simulink model "ACFT11_a_121"  (R2026a)
settings: Solver=ode15s  StopTime=2400  FixedStep=0.01  MaxStep=0.05  MinStep=1e-4  AbsTol=1e-4
model workspace (MAT data in the model file):
  op11 = opcond.OperatingPoint
  op11.Model_ = 'ACFT'
  op11.States_(1) = opcond.StatePoint
  op11.States_(1).Nx_ = 1
  op11.States_(1).Block_ = 'ACFT/EqM/BodyRates/p_radps'
  op11.States_(1).StateName_ = 'p_radps'
  op11.States_(1).x_ = -1.51786990083e-19
  op11.States_(2) = opcond.StatePoint
  op11.States_(2).Nx_ = 1
  op11.States_(2).Block_ = 'ACFT/EqM/BodyRates/q_radps'
  op11.States_(2).StateName_ = 'q_radps'
  op11.States_(2).x_ = 1.34070454591e-20
  op11.States_(3) = opcond.StatePoint
  op11.States_(3).Nx_ = 1
  op11.States_(3).Block_ = 'ACFT/EqM/BodyRates/r_radps'
  op11.States_(3).StateName_ = 'r_radps'
  op11.States_(3).x_ = 3.04056373945e-20
  op11.States_(4) = opcond.StatePoint
  op11.States_(4).Nx_ = 1
  op11.States_(4).Block_ = 'ACFT/EqM/BodyVelocities/u_mps'
  op11.States_(4).StateName_ = 'u_mps'
  op11.States_(4).x_ = 221.237928753
  op11.States_(5) = opcond.StatePoint
  op11.States_(5).Nx_ = 1
  op11.States_(5).Block_ = 'ACFT/EqM/BodyVelocities/v_mps'
  op11.States_(5).StateName_ = 'v_mps'
  op11.States_(5).x_ = -6.28259554611e-18
  op11.States_(6) = opcond.StatePoint
  op11.States_(6).Nx_ = 1
  op11.States_(6).Block_ = 'ACFT/EqM/BodyVelocities/w_mps'
  op11.States_(6).StateName_ = 'w_mps'
  op11.States_(6).x_ = 38.749469963
  op11.States_(7) = opcond.StatePoint
  op11.States_(7).Nx_ = 1
  op11.States_(7).Block_ = 'ACFT/EqM/EulerAngles/PHI_rad'
  op11.States_(7).StateName_ = 'PHI_rad'
  op11.States_(7).x_ = 1.38680229931e-18
  op11.States_(8) = opcond.StatePoint
  op11.States_(8).Nx_ = 1
  op11.States_(8).Block_ = 'ACFT/EqM/EulerAngles/PSI_rad'
  op11.States_(8).StateName_ = 'PSI_rad'
  op11.States_(8).x_ = -6.63244493967e-13
  op11.States_(9) = opcond.StatePoint
  op11.States_(9).Nx_ = 1
  op11.States_(9).Block_ = 'ACFT/EqM/EulerAngles/THETA_rad'
  op11.States_(9).StateName_ = 'THETA_rad'
  op11.States_(9).x_ = 0.17338965629
  op11.States_(10) = opcond.StatePoint
  op11.States_(10).Nx_ = 1
  op11.States_(10).Block_ = 'ACFT/EqM/InertialData/XI_m'
  op11.States_(10).StateName_ = 'XI_m'
  op11.States_(10).x_ = -1.46881201642e-12
  op11.States_(11) = opcond.StatePoint
  op11.States_(11).Nx_ = 1
  op11.States_(11).Block_ = 'ACFT/EqM/InertialData/YI_m1'
  op11.States_(11).StateName_ = 'YI_m'
  op11.States_(11).x_ = -2.21671166849e-12
  op11.States_(12) = opcond.StatePoint
  op11.States_(12).Nx_ = 1
  op11.States_(12).Block_ = 'ACFT/EqM/InertialData/ZI_m'
  op11.States_(12).StateName_ = 'ZI_m'
  op11.States_(12).x_ = -9997.44
  op11.Inputs_(1) = opcond.InputPoint
  op11.Inputs_(1).Block_ = 'ACFT/Elevator_deg'
  op11.Inputs_(1).PortWidth_ = 1
  op11.Inputs_(1).PortDimensions_ = [1 1]
  op11.Inputs_(1).u_ = -3.63207180524
  op11.Inputs_(2) = opcond.InputPoint
  op11.Inputs_(2).Block_ = 'ACFT/Aileron_deg'
  op11.Inputs_(2).PortWidth_ = 1
  op11.Inputs_(2).PortDimensions_ = [1 1]
  op11.Inputs_(2).u_ = 2.99398013712e-18
  op11.Inputs_(3) = opcond.InputPoint
  op11.Inputs_(3).Block_ = 'ACFT/Rudder_deg'
  op11.Inputs_(3).PortWidth_ = 1
  op11.Inputs_(3).PortDimensions_ = [1 1]
  op11.Inputs_(4) = opcond.InputPoint
  op11.Inputs_(4).Block_ = 'ACFT/Throttle'
  op11.Inputs_(4).PortWidth_ = 1
  op11.Inputs_(4).PortDimensions_ = [1 1]
  op11.Inputs_(4).u_ = 0.523236061228
  op_trim1 : opcond.OperatingReport (value not decoded)
  op_trim12 : opcond.OperatingReport (value not decoded)
  op_trim15 : opcond.OperatingReport (value not decoded)
  op_trim16 : opcond.OperatingReport (value not decoded)
  op_trim17 : opcond.OperatingReport (value not decoded)
  op_trim18 : opcond.OperatingReport (value not decoded)
  op_trim2 : opcond.OperatingReport (value not decoded)
  op_trim20 : opcond.OperatingReport (value not decoded)
  op_trim21 : opcond.OperatingReport (value not decoded)
  op_trim22 : opcond.OperatingReport (value not decoded)
  op_trim23 : opcond.OperatingReport (value not decoded)
  op_trim24 : opcond.OperatingReport (value not decoded)
  op_trim25 : opcond.OperatingReport (value not decoded)
  op_trim29 : opcond.OperatingReport (value not decoded)
  op_trim3 : opcond.OperatingReport (value not decoded)
  op_trim30 : opcond.OperatingReport (value not decoded)
  op_trim4 : opcond.OperatingReport (value not decoded)
  op_trim40 : opcond.OperatingReport (value not decoded)
  op_trim42 : opcond.OperatingReport (value not decoded)
  op_trim5 : opcond.OperatingReport (value not decoded)
  op_trim50 : opcond.OperatingReport (value not decoded)
  op_trim7 : opcond.OperatingReport (value not decoded)
  op_trim9 : opcond.OperatingReport (value not decoded)
values from neighbouring files (symbols this model uses):
  b = 9.05    [inertiatensor62.m]    (also in setup_bfl_analysis.m; setup_fcs_sim.m; setup_gschedule.m = geom.FCS_b; setup_takeoff_fcs.m)
  c = bar_colors{min(k,numel(bar_colors))}    [analyze_bfl.m]    (also in inertiatensor62.m = 15.55; optimize_indi_gains.m = 15.55; restore_normal_fcs.m = 15.55; run_bfl_sweep.m = 15.55)
  CL_AlphaDot = 0    [inertiatensor62.m]    (also in setup_bfl_analysis.m; setup_fcs_sim.m; setup_takeoff_fcs.m)
  Cm_AlphaDot = 0    [inertiatensor62.m]    (also in setup_bfl_analysis.m; setup_fcs_sim.m; setup_takeoff_fcs.m)
  FCS_aerospike_thrust = 250000.0    (= 250000)    [fcs_params.m]
  FCS_alpha_max = 16.0    (= 16)    [fcs_params.m]
  FCS_bank_max = 45.0    (= 45)    [fcs_params.m]
  FCS_da_max = 20.0    (= 20)    [fcs_params.m]
  FCS_de_max = 25.0    (= 25)    [fcs_params.m]
  FCS_dr_max = 25.0    (= 25)    [fcs_params.m]
  FCS_dt = 0.01    [fcs_params.m]
  FCS_g = 9.80665    [fcs_params.m]
  FCS_Gmin_p = 0.02    [fcs_params.m]
  FCS_Gmin_q = 0.02    [fcs_params.m]
  FCS_Gmin_r = 0.01    [fcs_params.m]
  FCS_h_gnd = 2.24    [fcs_params.m]
  FCS_hdot_max = 30.0    (= 30)    [fcs_params.m]
  FCS_hdot_td = 0.3    [fcs_params.m]
  FCS_Kalpha = 3.0    (= 3)    [fcs_params.m]
  FCS_Kalpha_lim = 2.0    (= 2)    [fcs_params.m]
  FCS_Kbeta = 2.0    (= 2)    [fcs_params.m]
  FCS_Kflare = 1.0    (= 1)    [fcs_params.m]
  FCS_Kgamma = 1.5    [fcs_params.m]
  FCS_Kh = 0.10    (= 0.1)    [fcs_params.m]
  FCS_Knz = 20.0    (= 20)    [fcs_params.m]
  FCS_Kp = 6.0    (= 6)    [fcs_params.m]
  FCS_Kphi = 3.0    (= 3)    [fcs_params.m]
  FCS_Kq = 5.0    (= 5)    [fcs_params.m]
  FCS_Kr = 4.0    (= 4)    [fcs_params.m]
  FCS_Ktheta = 2.0    (= 2)    [fcs_params.m]
  FCS_link_timeout = 1.0    (= 1)    [fcs_params.m]
  FCS_MODE_AUTO = 0    [fcs_params.m]
  FCS_Nfilt = 20.0    (= 20)    [fcs_params.m]
  FCS_Nz_max = 3.0    (= 3)    [fcs_params.m]
  FCS_Nz_min = -1.0    (= -1)    [fcs_params.m]
  FCS_p_max = 60.0    (= 60)    [fcs_params.m]
  FCS_q_max = 15.0    (= 15)    [fcs_params.m]
  FCS_qbar_hi = 6000.0    (= 6000)    [fcs_params.m]
  FCS_qbar_lo = 1000.0    (= 1000)    [fcs_params.m]
  FCS_r_max = 15.0    (= 15)    [fcs_params.m]
  FCS_relight_M_hi = 2.0    (= 2)    [fcs_params.m]
  FCS_relight_M_lo = 0.35    [fcs_params.m]
  FCS_relight_qbar = 3000.0    (= 3000)    [fcs_params.m]
  FCS_stick_detent = 0.03    [fcs_params.m]
  FCS_stick_p_scale = 60.0    (= 60)    [fcs_params.m]
  FCS_stick_q_scale = 15.0    (= 15)    [fcs_params.m]
  FCS_tau_flare = 8.0    (= 8)    [fcs_params.m]
  FCS_TECS_Kep = 0.25    [fcs_params.m]
  FCS_TECS_Ktp = 0.30    (= 0.3)    [fcs_params.m]
  FCS_theta_climb = 12.0    (= 12)    [fcs_params.m]
  FCS_theta_max = 30.0    (= 30)    [fcs_params.m]
  FCS_theta_min = -20.0    (= -20)    [fcs_params.m]
  FCS_theta_trim = 0.0    (= 0)    [fcs_params.m]
  FCS_thr_max = 1.0    (= 1)    [fcs_params.m]
  FCS_thr_min = 0.0    (= 0)    [fcs_params.m]
  FCS_thr_trim = 0.50    (= 0.5)    [fcs_params.m]
  FCS_V_rotate = 94.0    (= 94)    [fcs_params.m]
  FCS_Vmin = 60.0    (= 60)    [fcs_params.m]
  FF_rates = [0.0,              2.5,              5.0,             73.0,             78.0,              0.5]    [fcs_params.m]
  g = 9.80665    [inertiatensor62.m]    (also in setup_bfl_analysis.m; setup_fcs_sim.m; setup_takeoff_fcs.m)
  GS_Gp_tab = Cl_da * (S*b/Ixx)    [setup_gschedule.m]
  GS_Gq_tab = Cm_de * (S*c/Iyy)    [setup_gschedule.m]
  GS_Gr_tab = Cn_dr * (S*b/Izz)    [setup_gschedule.m]
  MASS_fuel_total = MASS_full - MASS_empty - MASS_orbiter    (= 14700)    [fcs_params.m]
  S = 85.25    [inertiatensor62.m]    (also in optimize_indi_gains.m; restore_normal_fcs.m; run_bfl_sweep.m; setup_bfl_analysis.m)
  s = [s, sprintf(' ... (first row only)    [setup_propulsion.m]
  y_cg = 0    [inertiatensor62.m]    (also in setup_bfl_analysis.m; setup_fcs_sim.m; setup_takeoff_fcs.m)
  z_cg = 0.0    (= 0)    [inertiatensor62.m]    (also in setup_bfl_analysis.m; setup_fcs_sim.m; setup_takeoff_fcs.m)
undefined symbols (not defined in the file or in its folder): deg, DiscIntNeverNeededParam, EqM, GS_alpha_cl, GS_alpha_cm, GS_alpha_cn, GS_mach_cl, GS_mach_cm, GS_mach_cn, rad
libraries: aerolibconvert2 x21, simulink x7, aerolibfltsims x3, aerolibanim x1, aerolibatmos2 x1, shareddyn x1
(part 1 of 4)
settings Model: PacingRate=20  Creator=bruno  LastModifiedBy=tejve
settings SolverCC: MaxConsecutiveMinStep=3  ZeroCrossAlgorithm=Adaptive  EnableFixedStepZeroCrossing=on
settings DataIOCC: ExternalInput=takeoff_u  InitialState=getstatestruct(op_trim1)
settings DebuggingCC: MinStepSizeMsg=error  MaskedZcDiagnostic=none  IgnoredZcDiagnostic=none  UnderSpecifiedDimensionMsg=warning

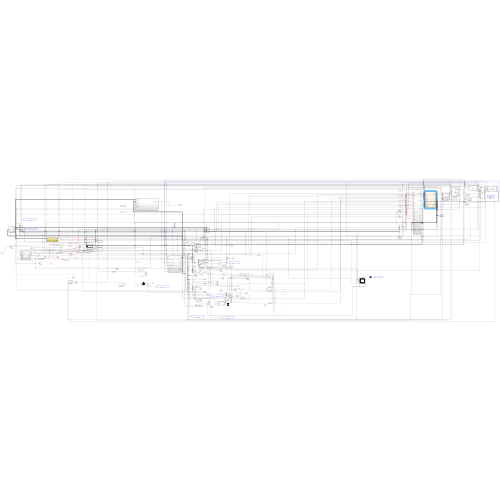
[thumbnail: Simulink's stored preview of the top-level diagram]
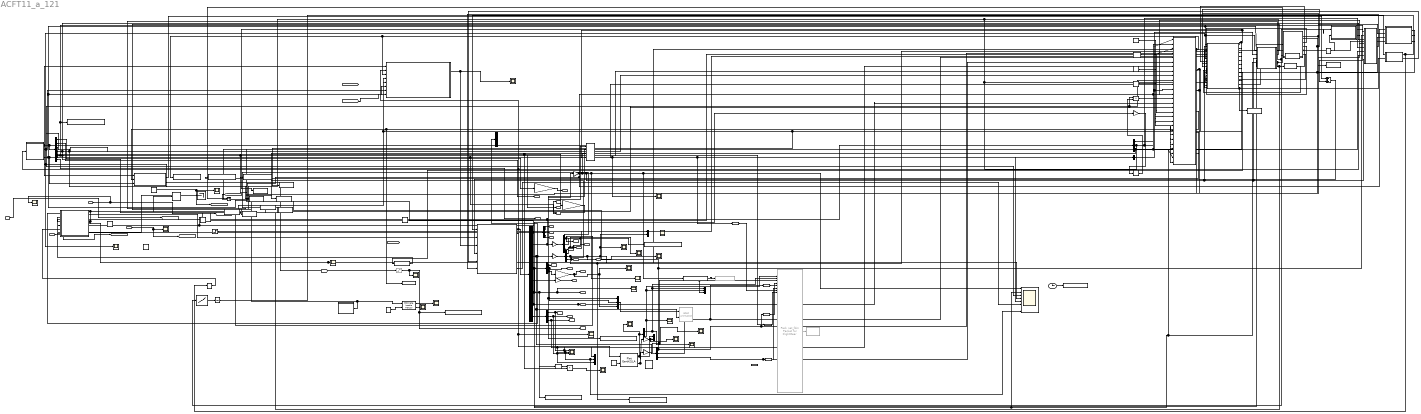
== system ACFT11_a_121 ==
  Elevator_deg : Inport  OutDataTypeStr=double
  Aileron_deg : Inport  Port=2  OutDataTypeStr=double
  Rudder_deg : Inport  Port=3  OutDataTypeStr=double
  Throttle : Inport  Port=4  OutDataTypeStr=double
  6DoF Animation : aerolibanim/6DoF Animation  Commented=on  u1=[0 40000 -20000 20000 -50000 -30000]  u2=0.1  u3=400  u4=[0 0 0]  u5=Fly alongside  u6=[10000 10000 10000]  u7=9  u8=on
  Aerospike : MATLAB Function  TreatAsAtomicUnit=on
  Aerospike_Tmax : Constant  Value=FCS_aerospike_thrust
  Aerovegamidfid : Subsystem  AncestorBlock=Aerodynamic/Aero
  Alt_1000m_trigger : simulink/Logic and Bit Operations/Compare To Constant  relop=>=  const=9999  OutDataTypeStr=boolean
  Angle Conversion : aerolibconvert2/Angle Conversion  IU=deg  OU=rad
  Atmospheric : Subsystem  AncestorBlock=Atmospheric/Atmospheric
  Bus Selector : BusSelector  OutputSignals=CAS_mps,Mach,TAS_mps,Beta_deg,Alpha_deg,AlphaDot_radps
  Bus Selector1 : BusSelector  OutputSignals=VB_mps,BodyRates_radps,EulerAngles_rad,IntertialPosition_m,GroundSpeed_mps,Gamma_deg,Track_deg,LoadFactors
  Cg AS PERCENTGE OF TOTAL LENGTH CREF : Constant  Value=0.6168
  Clock_FCS : Clock
  Constant : Constant  Value=[0,0,0,0,0,0]
  Constant1 : Constant
  Constant2 : Constant  Value=1.2
  Constant3 : Constant  Value=0
  Constant4 : Constant  Value=0
  Data Type Conversion{,1..4,8} (6 alike) : DataTypeConversion  OutDataTypeStr=single  SaturateOnIntegerOverflow=off  RndMeth=Floor
  Demux{,1..5,10} (7 alike) : Demux  Outputs=3
  Demux6 : Demux  Outputs=2
  DtcDesc : DataTypeConversion  OutDataTypeStr=double  SaturateOnIntegerOverflow=off  RndMeth=Floor
  DtcRl : DataTypeConversion  OutDataTypeStr=double  SaturateOnIntegerOverflow=off  RndMeth=Floor
  EqM : Subsystem  AncestorBlock=EqM/EqM
  Estimate Inertia Tensor : shareddyn/Estimate Inertia Tensor  fmass=28500  emass=10800  fI=Inertia  eI=InertiaEmpty  aMode=aMode
      settings: LibrarySourceBlock=|
      | aerolibbdyn/Estimate
      | Inertia Tensor
  Estimation : Subsystem
  FCS : Subsystem
  FCS_RC_age : Constant  Value=0
  FCS_RC_mode : Constant  Value=FCS_MODE_AUTO
  FCS_RC_pitch : Constant  Value=0
  FCS_RC_roll : Constant  Value=0
  FCS_Vz_calc : Product  Inputs=**
  FCS_gamma_d2r : Gain  Gain=pi/180
  FCS_rate_demux : Demux  Outputs=3
  FCS_rho_sel : BusSelector  OutputSignals=rho_kgpm3
  FCS_sin_gamma : Trigonometry
  FfLut : Lookup_n-D  NumberOfTableDimensions=1  BreakpointsForDimension1=[0 1 2 3 4 5]  Table=FF_rates  InterpMethod=Flat  ExtrapMethod=Clip  InternalRulePriority=Speed  RndMeth=Simplest
  Flat Earth to LLA : FlatEarth2LLA  R=6378137  LL0=[36.973889000000000 -25.171111000000000]
  FuelInt : Integrator  UpperSaturationLimit=MASS_fuel_total  LowerSaturationLimit=0
  Gain : Gain
  Gain1 : Gain  Gain=-1
  Gain2 : Gain  Gain=-1
  Generate Run Script1 : aerolibfltsims/Generate Run Script  Architecture=Win64  dataFlow=Send  GeometryModelName=c172p  AirportId=1  RunwayId=1  InitialAltitude=0  InitialHeading=0  OffsetDistance=0  OffsetAzimuth=0  InstallScenery=off  DisableShaders=off  OriginAddress=127.0.0.1  DestinationPort=5502  OriginPort=5505  LocalAddress=127.0.0.1  OutputFileName=tj112.bat  FlightGearBaseDirectory=C:\Program Files\FlightGear 2020.3.2
  GlideCompute : MATLAB Function  TreatAsAtomicUnit=on
  Landing Gear : Subsystem
  ManeuverScope : Scope  NumInputPorts=8
      settings: ActiveDisplayString=8  ActiveDisplayYMinimum=-2.289254531971836  ActiveDisplayYMaximum=5.0402128679995908  DataLoggingVariableName=ScopeData55
  MassModel : MATLAB Function  TreatAsAtomicUnit=on
  MemMass : Memory  InitialCondition=28500
  MissionManager : Stateflow chart  TreatAsAtomicUnit=on
  Mux : Mux  Inputs=2
  Mux1 : Mux  Inputs=3
  Mux3 : Mux  Inputs=3
  Mux4 : Mux  Inputs=2
  Mux7 : Mux  Inputs=3
  Nf_LiftoffScope : Scope
  Pack net_fdm Packet for FlightGear : aerolibfltsims/Pack net_fdm Packet for FlightGear  Commented=on  FlightGearVersion=v2019.1  ShowPositionAttitudeInputs=on  ShowVelocityAccelerationInputs=on  ShowControlSurfacePositionInputs=on  ShowEngineFuelInputs=on  ShowLandingGearInputs=off  ShowEnvironmentInputs=off  SampleTime=-1  packetVersion=24
  Product : Product
  Propulsion : Subsystem  AncestorBlock=Propulsion/Propulsion
  RCS_ctrl : MATLAB Function  TreatAsAtomicUnit=on
  RTB_Guidance : MATLAB Function  TreatAsAtomicUnit=on
  Saturation2 : Saturate  Commented=through  UpperLimit=250000  LowerLimit=0
  Scope{,1..7,10..14,18,20} (15 alike) : Scope
      Scope settings: ActiveDisplayYMinimum=-13.152364949660917  ActiveDisplayYMaximum=60.1028018218888  YLabel=Flight path angle(deg)  DataLoggingVariableName=ScopeData5
      Scope1 settings: ActiveDisplayYMinimum=-1  ActiveDisplayYMaximum=1
      Scope10 settings: ActiveDisplayYMinimum=0.61360792662227759  ActiveDisplayYMaximum=0.63379776950955791  DataLoggingVariableName=ScopeData11
      Scope11 settings: ActiveDisplayYMinimum=-1340.90587  ActiveDisplayYMaximum=11603.05287  DataLoggingVariableName=ScopeData12
      Scope12 settings: ActiveDisplayYMinimum=-623.957  ActiveDisplayYMaximum=5615.613  DataLoggingVariableName=ScopeData13
      Scope13 settings: ActiveDisplayYMinimum=-1  ActiveDisplayYMaximum=1
      Scope14 settings: ActiveDisplayYMinimum=-1.0801678452245245  ActiveDisplayYMaximum=10.282171182560381  DataLoggingVariableName=ScopeData21
      Scope18 settings: ActiveDisplayYMinimum=-1  ActiveDisplayYMaximum=1  DataLoggingVariableName=ScopeData29
      Scope2 settings: ActiveDisplayYMinimum=-1  ActiveDisplayYMaximum=1  DataLoggingVariableName=ScopeData2
      Scope20 settings: ActiveDisplayYMinimum=0.90512395677267277  ActiveDisplayYMaximum=2.9051239567726728  DataLoggingVariableName=ScopeData31
      Scope3 settings: ActiveDisplayYMinimum=-1  ActiveDisplayYMaximum=1  DataLoggingVariableName=ScopeData3
      Scope4 settings: ActiveDisplayYMinimum=-10822.330699949573  ActiveDisplayYMaximum=8964.1397199268285
      Scope5 settings: ActiveDisplayYMinimum=2.6766585887324741  ActiveDisplayYMaximum=69.223535186339291
      Scope6 settings: ActiveDisplayYMinimum=-1.0137729913835152  ActiveDisplayYMaximum=70.044552754707041  DataLoggingVariableName=ScopeData22
      Scope7 settings: ActiveDisplayYMinimum=-35300.079820700717  ActiveDisplayYMaximum=108949.5506916134  DataLoggingVariableName=ScopeData23
  Send net_fdm Packet to FlightGear : aerolibfltsims/Send net_fdm Packet to FlightGear  Commented=on  DestinationIpAddress=127.0.0.1  DestinationPort=5502  LocalIpPort=-1  varLen=off  SampleTime=-1
  Stop_at_1000m : Stop  Commented=on
  TW_Alpha_deg : ToWorkspace  VariableName=TW_Alpha_deg  SampleTime=0.1
  TW_E_spec : ToWorkspace  VariableName=TW_E_spec  SaveFormat=Timeseries  SampleTime=-1
  TW_Gamma_deg : ToWorkspace  VariableName=TW_Gamma_deg  SampleTime=0.1
  TW_Mach : ToWorkspace  VariableName=Machlog  SaveFormat=Timeseries  SampleTime=-1
  TW_MissionPhase : ToWorkspace  VariableName=TW_MissionPhase  SaveFormat=Timeseries  SampleTime=-1
  TW_Ntotal : ToWorkspace  VariableName=TW_Ntotal  SampleTime=0.02
  TW_Phase : ToWorkspace  VariableName=TW_Phase  SampleTime=-1
  TW_TAS_mps : ToWorkspace  VariableName=TW_TAS_mps  SampleTime=0.1
  TW_T_aero : ToWorkspace  VariableName=T_aero  SaveFormat=Timeseries  SampleTime=-1
  TW_Theta_deg : ToWorkspace  VariableName=TW_Theta_deg  SampleTime=0.1
  TW_Throttle : ToWorkspace  VariableName=TW_Throttle  SampleTime=0.02
  TW_Thrust_N : ToWorkspace  VariableName=TW_Thrust_N  SampleTime=0.1
  TW_V : ToWorkspace  VariableName=Vlog  SaveFormat=Timeseries  SampleTime=-1
  TW_Vz_est : ToWorkspace  VariableName=TW_Vz_est  SaveFormat=Timeseries  SampleTime=-1
  TW_X_m : ToWorkspace  VariableName=TW_X_m  SampleTime=0.1
  TW_ail : ToWorkspace  VariableName=TW_ail  SaveFormat=Timeseries  SampleTime=-1
  TW_al : ToWorkspace  VariableName=al_log  SaveFormat=Timeseries  SampleTime=-1
  TW_beta : ToWorkspace  VariableName=TW_beta  SaveFormat=Timeseries  SampleTime=-1
  TW_beta2 : ToWorkspace  VariableName=beta_log  SaveFormat=Timeseries  SampleTime=-1
  TW_brg : ToWorkspace  VariableName=brg_log  SaveFormat=Timeseries  SampleTime=-1
  TW_da : ToWorkspace  VariableName=da_log  SaveFormat=Timeseries  SampleTime=-1
  TW_de : ToWorkspace  VariableName=de_log  SaveFormat=Timeseries  SampleTime=-1
  TW_dr2 : ToWorkspace  VariableName=dr_log  SaveFormat=Timeseries  SampleTime=-1
  TW_elev_cmd : ToWorkspace  VariableName=TW_elev_cmd  SampleTime=-1
  TW_h : ToWorkspace  VariableName=hlog  SaveFormat=Timeseries  SampleTime=-1
  TW_p : ToWorkspace  VariableName=TW_p  SaveFormat=Timeseries  SampleTime=-1
  TW_phase : ToWorkspace  VariableName=phase  SaveFormat=Timeseries  SampleTime=-1
  TW_phi : ToWorkspace  VariableName=phi_log  SaveFormat=Timeseries  SampleTime=-1
  TW_posNED : ToWorkspace  VariableName=TW_posNED  SampleTime=0.02
  TW_prop_mode : ToWorkspace  VariableName=prop_mode  SaveFormat=Timeseries  SampleTime=-1
  TW_psi : ToWorkspace  VariableName=TW_psi  SaveFormat=Timeseries  SampleTime=-1
  TW_q : ToWorkspace  VariableName=q_log2  SaveFormat=Timeseries  SampleTime=-1
  TW_q_deg : ToWorkspace  VariableName=TW_q_deg  SampleTime=0.1
  TW_qbar : ToWorkspace  VariableName=TW_qbar  SaveFormat=Timeseries  SampleTime=-1
  TW_qcmd : ToWorkspace  VariableName=TW_qcmd  SampleTime=-1
  TW_r : ToWorkspace  VariableName=TW_r  SaveFormat=Timeseries  SampleTime=-1
  TW_r2 : ToWorkspace  VariableName=r_log  SaveFormat=Timeseries  SampleTime=-1
  TW_relight_ok : ToWorkspace  VariableName=TW_relight_ok  SaveFormat=Timeseries  SampleTime=-1
  TW_rng : ToWorkspace  VariableName=rng_log  SaveFormat=Timeseries  SampleTime=-1
  TW_rud : ToWorkspace  VariableName=TW_rud  SaveFormat=Timeseries  SampleTime=-1
  TW_sep_cmd : ToWorkspace  VariableName=sep_cmd  SaveFormat=Timeseries  SampleTime=-1
  TW_time : ToWorkspace  VariableName=TW_time  SampleTime=0.1
  TW_trk : ToWorkspace  VariableName=trk_log  SaveFormat=Timeseries  SampleTime=-1
  Term_NGears : Terminator
  Thrust : Scope
      settings: ActiveDisplayYMinimum=-1.0708895352839015E+7  ActiveDisplayYMaximum=1.709230025160585E+8  DataLoggingVariableName=ScopeData4
  ThrustSum : Sum
  Traj3D : MATLAB Function  TreatAsAtomicUnit=on
  Vr_cmd : Constant  Value=FCS_V_rotate
  aerospike : Subsystem
  alpha : Scope
      settings: ActiveDisplayYMinimum=-224.99999999838857  ActiveDisplayYMaximum=224.99999998795374  YLabel=Alpha(deg)  DataLoggingVariableName=ScopeData4
  altitude feet : Scope
      settings: ActiveDisplayYMinimum=-16310.123094954164  ActiveDisplayYMaximum=161835.60391679878
  altitudem : Scope
      settings: ActiveDisplayYMinimum=-1  ActiveDisplayYMaximum=1  DataLoggingVariableName=ScopeData32
  begin_descent_cmd : Step  Time=400  SampleTime=0
  ias : Scope
      settings: ActiveDisplayYMinimum=-111.24738835049642  ActiveDisplayYMaximum=1011.226495154468  DataLoggingVariableName=ScopeData2
  lattitude : Scope
      settings: ActiveDisplayYMinimum=37.605975805600643  ActiveDisplayYMaximum=37.625326099444457  DataLoggingVariableName=ScopeData28
  load factor : Scope  NumInputPorts=3
      settings: ActiveDisplayYMinimum=-0.60668568177734672  ActiveDisplayYMaximum=4.4635157428572985
  longitude : Scope
      settings: ActiveDisplayYMinimum=-25.133530310627574  ActiveDisplayYMaximum=-25.13229966034443  DataLoggingVariableName=ScopeData30
  m2ft : Gain  Gain=-1/0.3048
  mps2kt : Gain  Gain=1/0.51444444
  mps2kt1 : Gain  Gain=1/0.51444444
  mps2kt2 : Gain  Gain=1/0.51444444
  mu_cmd_Memory : Memory  InitialCondition=0.03  InheritSampleTime=on
  rad2deg : Gain  Gain=180/pi
  rad2deg1 : Gain  Gain=180/pi
  term_desc : Terminator
  term_gear : Terminator
  theta : Scope
      settings: Title=Theta  ActiveDisplayYMinimum=-10.965778597195566  ActiveDisplayYMaximum=61.928191508155521  YLabel=Theta(deg)
  KCAS : Outport
  Mach : Outport  Port=2
  KTAS : Outport  Port=3
  Beta_deg : Outport  Port=4
  Alpha_deg : Outport  Port=5
  AlphaDot_radps : Outport  Port=6
  u_mps : Outport  Port=7
  v_mps : Outport  Port=8
  w_mps : Outport  Port=9
  p_radps : Outport  Port=10
  q_radps : Outport  Port=11
  r_radps : Outport  Port=12
  Phi_deg : Outport  Port=13
  Theta_deg : Outport  Port=14
  Psi_deg : Outport  Port=15
  X_m : Outport  Port=16
  Y_m : Outport  Port=17
  PresAlt_ft : Outport  Port=18
  GSpeed_kt : Outport  Port=19
  Gamma_deg : Outport  Port=20
  Track_deg : Outport  Port=21
  nx : Outport  Port=22
  ny : Outport  Port=23
  nz : Outport  Port=24
  Thrust_N : Outport  Port=25
  wires:
  Cg AS PERCENTGE OF TOTAL LENGTH CREF/1 -> [CG_mac], Scope10/1
  [CG_mac] -> Aerovegamidfid/6(CG_mac)
  mps2kt/1 -> KCAS/1
  mps2kt1/1 -> KTAS/1
  Demux/1 -> u_mps/1
  Demux/2 -> v_mps/1
  Demux/3 -> w_mps/1
  Demux1/1 -> p_radps/1, TW_p/1
  Demux1/3 -> r_radps/1, TW_r/1
  Demux2/1 -> Scope2/1, Mux/1, Phi_deg/1
  Demux2/3 -> TW_psi/1, Scope3/1, Psi_deg/1
  rad2deg/1 -> Demux1/1
  rad2deg1/1 -> Demux2/1
  m2ft/1 -> PresAlt_ft/1, altitude feet/1, Mux1/3
  Bus Selector1/5 -> mps2kt2/1  "<GroundSpeed_mps>"
  mps2kt2/1 -> GSpeed_kt/1
  Bus Selector1/7 -> FCS/15(track_deg), Track_deg/1, TW_trk/1  "<Track_deg>"
  Bus Selector1/8 -> Demux5/1  "<LoadFactors>"
  Demux5/1 -> Mux7/1, load factor/1, nx/1  "nx"
  Demux5/2 -> Mux7/3, load factor/3, ny/1  "ny"
  Mux1/1 -> 6DoF Animation/1
  Demux4/1 -> RCS_ctrl/2(phi_rad), TW_phi/1, FCS/4(phi_rad), Data Type Conversion/1
  Demux4/2 -> FCS/5(theta_rad), Data Type Conversion1/1
  Demux4/3 -> FCS/6(psi_rad), Data Type Conversion2/1
  Constant4/1 -> Flat Earth to LLA/2
  Pack net_fdm Packet for FlightGear/1 -> Send net_fdm Packet to FlightGear/1
  Angle Conversion/1 -> Product/1
  Product/1 -> Scope5/1
  Data Type Conversion/1 -> Pack net_fdm Packet for FlightGear/4
  Data Type Conversion1/1 -> Pack net_fdm Packet for FlightGear/5
  Data Type Conversion2/1 -> Pack net_fdm Packet for FlightGear/6
  Data Type Conversion3/1 -> Pack net_fdm Packet for FlightGear/7
  Data Type Conversion4/1 -> Pack net_fdm Packet for FlightGear/8
  Throttle/1 -> [Throttle], Scope14/1
  aerospike/1(net mass) -> Estimate Inertia Tensor/1, [Mass_kg]
  Estimate Inertia Tensor/2 -> Scope12/1
  Gain/1 -> Pack net_fdm Packet for FlightGear/3, Mux3/3, Scope1/1
  Elevator_deg/1 -> [Elevator_deg], Scope20/1
  ? -> ?
  Demux5/3 -> nz/1, ManeuverScope/8, Mux7/2, load factor/2, FCS/7(Nz_g)  "Normal LoadFactor"
  Constant3/1 -> Estimate Inertia Tensor/2
  Bus Selector1/1 -> Demux/1, Landing Gear/2(VB_mps)  "<VB_mps>"
  Bus Selector1/4 -> RTB_Guidance/1(pos_NED), TW_posNED/1, Landing Gear/4(pos_NED_m), Demux3/1  "<IntertialPosition_m>"
  Landing Gear/3(N_gears_N) -> Term_NGears/1
  Aileron_deg/1 -> [Aileron_deg]
  Propulsion/2(Thrust_N) -> Saturation2/1
  Alt_1000m_trigger/1 -> Stop_at_1000m/1
  Rudder_deg/1 -> [Rudder_deg]
  Bus Selector1/2 -> FCS_rate_demux/1, Landing Gear/3(BodyRates_radps), rad2deg/1  "<BodyRates_radps>"
  Landing Gear/2(N_total_N) -> Nf_LiftoffScope/1, MissionManager/3(Ngear), FCS/16(Ngear_N), TW_Ntotal/1
  Bus Selector1/3 -> Demux4/1, 6DoF Animation/2, rad2deg1/1, Demux10/1, Landing Gear/1(EulerAngles_rad)  "<EulerAngles_rad>"
  Bus Selector/5 -> TW_al/1, FCS/8(alpha_deg), RCS_ctrl/1(alpha_deg), TW_Alpha_deg/1, Data Type Conversion3/1, ManeuverScope/5, alpha/1, Alpha_deg/1  "<Alpha_deg>"
  Demux1/2 -> q_radps/1, TW_q_deg/1
  Saturation2/1 -> TW_Thrust_N/1, Thrust_N/1, Thrust/1
  Gain1/1 -> Mux4/2, Scope18/1
  Flat Earth to LLA/2 -> Gain/1, Gain1/1
  Demux6/2 -> Pack net_fdm Packet for FlightGear/1, Mux3/2, longitude/1  "longitude"
  Demux6/1 -> Pack net_fdm Packet for FlightGear/2, Mux3/1, lattitude/1  "lattitude"
  Flat Earth to LLA/1 -> Demux6/1, Scope6/1, Mux4/1
  Demux2/2 -> MissionManager/4(theta), TW_Theta_deg/1, Mux/2, theta/1, ManeuverScope/4, Theta_deg/1  "theta"
  Bus Selector1/6 -> Estimation/4(gamma_deg), FCS/27(gamma_deg), ManeuverScope/2, FCS_gamma_d2r/1, Gamma_deg/1, Scope/1, Angle Conversion/1, TW_Gamma_deg/1  "<Gamma_deg>"
  Bus Selector/6 -> AlphaDot_radps/1  "<AlphaDot_radps>"
  Bus Selector/4 -> RCS_ctrl/3(beta_deg), TW_beta2/1, FCS/9(beta_deg), TW_beta/1, Beta_deg/1, Data Type Conversion4/1  "<Beta_deg>"
  Bus Selector/3 -> mps2kt1/1, Product/2  "<TAS_mps>"
  Bus Selector/2 -> Mach/1  "<Mach>"
  Bus Selector/1 -> mps2kt/1  "<CAS_mps>"
  Estimate Inertia Tensor/1 -> Scope11/1
  Clock_FCS/1 -> TW_time/1
  mu_cmd_Memory/1 -> Landing Gear/6(mu_cmd)
  FCS_gamma_d2r/1 -> FCS_sin_gamma/1
  FCS_sin_gamma/1 -> FCS_Vz_calc/2
  FCS_rate_demux/1 -> RCS_ctrl/4(p), FCS/1(p_radps)
  FCS_rate_demux/2 -> RCS_ctrl/5(q), FCS/2(q_radps), TW_q/1
  FCS_rate_demux/3 -> RCS_ctrl/6(r), FCS/3(r_radps), TW_r2/1
  FCS_rho_sel/1 -> Estimation/2(rho), FCS/12(rho_kgpm3)  "<rho_kgpm3>"
  FCS_Vz_calc/1 -> FCS/14(Vz_mps)
  FCS_RC_mode/1 -> FCS/17(RC_mode)
  FCS_RC_pitch/1 -> FCS/18(RC_pitch)
  FCS_RC_roll/1 -> FCS/19(RC_roll)
  FCS_RC_age/1 -> FCS/20(RC_cmd_age)
  FCS/1(Elevator_deg) -> TW_elev_cmd/1, Aerovegamidfid/3(Elevator_deg), TW_de/1
  FCS/2(Aileron_deg) -> TW_ail/1, Aerovegamidfid/4(Aileron_deg), TW_da/1
  FCS/3(Rudder_deg) -> TW_rud/1, Aerovegamidfid/5(Rudder_deg), TW_dr2/1
  FCS/4(Throttle) -> TW_Throttle/1, Propulsion/2(Throttle)
  FCS/5(Mode_out) -> TW_Phase/1
  FCS/6(q_cmd_deg_s) -> TW_qcmd/1
  Atmospheric/1(FromAtmos) -> FCS_rho_sel/1, Bus Selector/1, Propulsion/1(FromAtmos), Aerovegamidfid/1(From Atmos)  "FromAtmos"
  Atmospheric/4(mach) -> TW_Mach/1, MissionManager/7(Mach), Estimation/5(mach), Aerovegamidfid/8(mach), FCS/11(Mach), Propulsion/3(Mach)
  Atmospheric/2(TAS_mps) -> TW_V/1, ias/1, Estimation/1(V), MissionManager/1(V), FCS/10(V_mps), FCS_Vz_calc/1, Aerovegamidfid/7(TAS_mps), ManeuverScope/3, TW_TAS_mps/1  "Airspeed"
  Vr_cmd/1 -> MissionManager/5(Vr)
  MissionManager/2(law_select) -> FCS/24(law_select)
  MissionManager/3(V_cmd) -> FCS/21(V_cmd)
  MissionManager/4(h_cmd) -> FCS/22(h_cmd)
  MissionManager/5(psi_cmd) -> FCS/23(psi_cmd)
  MissionManager/6(q_rot_cmd) -> FCS/25(q_rot_cmd)
  MissionManager/7(thr_cmd) -> FCS/26(thr_cmd)
  MissionManager/8(brake_cmd) -> mu_cmd_Memory/1
  MissionManager/9(gear_cmd) -> term_gear/1
  begin_descent_cmd/1 -> MissionManager/6(begin_descent)
  Estimation/1(E_spec) -> TW_E_spec/1
  Estimation/2(qbar) -> RCS_ctrl/7(qbar), MissionManager/11(qbar), TW_qbar/1
  Estimation/3(Vz) -> TW_Vz_est/1
  RTB_Guidance/1(range_home) -> GlideCompute/2(range_home), MissionManager/9(range_home), TW_rng/1
  RTB_Guidance/2(bearing_home) -> GlideCompute/3(bearing_home), TW_brg/1, MissionManager/10(bearing_home)
  MissionManager/10(gamma_cmd) -> FCS/28(gamma_cmd)
  MissionManager/11(prop_mode) -> FfLut/1, Aerospike/1(prop_mode), TW_prop_mode/1
  Propulsion/1(Engine_Forces_and Moments) -> ThrustSum/1
  Aerospike/1(F6) -> ThrustSum/2
  Aerospike_Tmax/1 -> Aerospike/2(T_max)
  Aerospike/2(T_aero) -> TW_T_aero/1
  MissionManager/1(phase) -> TW_MissionPhase/1, Traj3D/4(phase), TW_phase/1
  Demux3/1 -> Mux1/1, TW_X_m/1, Traj3D/1(N), X_m/1
  Demux3/2 -> Y_m/1, Mux1/2, Traj3D/2(E)
  Demux3/3 -> m2ft/1, Gain2/1
  Gain2/1 -> GlideCompute/1(h), TW_h/1, Estimation/3(alt), RCS_ctrl/8(h), MissionManager/2(h), Alt_1000m_trigger/1, ManeuverScope/1, altitudem/1, Traj3D/3(alt), FCS/13(alt_m)  "altitudem"
  FfLut/1 -> FuelInt/1
  FuelInt/1 -> MassModel/1(fuel_burned)
  RTB_Guidance/5(gs_alt_cmd) -> GlideCompute/4(gs_alt_cmd), MissionManager/15(gs_alt_cmd)
  RTB_Guidance/3(xtrack_err) -> MissionManager/13(xtrack_err)
  RTB_Guidance/4(along_track) -> MissionManager/14(along_track)
  RTB_Guidance/6(loc_hdg_cmd) -> MissionManager/16(loc_hdg_cmd)
  GlideCompute/1(glide_gamma_cmd) -> MissionManager/17(glide_gamma_cmd)
  GlideCompute/2(glide_psi_cmd) -> MissionManager/18(glide_psi_cmd)
  GlideCompute/3(app_h_cmd) -> MissionManager/19(app_h_cmd)
  MemMass/1 -> Landing Gear/5(mass_kg)
  MassModel/2(Inertia) -> EqM/5(InertiaTensor_kgm2)
  MassModel/1(mass_kg) -> MemMass/1, EqM/1(Mass_kg)
  RCS_ctrl/1(F6) -> EqM/6(RCS_cmd)
  ThrustSum/1 -> EqM/4(ThrustForcesMoments_N_Nm)
  EqM/1(EqM) -> Aerovegamidfid/2(FromEqM), Atmospheric/1(FromEqM), Bus Selector1/1  "FromEqM"
  EqM/2(inp) -> Flat Earth to LLA/1, Scope7/1
  Landing Gear/1(GndForces_N_Nm) -> EqM/2(GroundForcesMoments_N_Nm)
  EqM/11(verticalvelocity) -> ManeuverScope/6  "Vertical Velocity"
  Aerovegamidfid/1(AeroForcesMoments) -> Scope4/1, EqM/3(AeroForcesMoments_N_Nm)
  DtcRl/1 -> MissionManager/8(relight_ok)
  MissionManager/12(sep_cmd) -> MassModel/2(sep_cmd), TW_sep_cmd/1
  Estimation/5(relight_ok) -> DtcRl/1, TW_relight_ok/1
  DtcDesc/1 -> MissionManager/12(descending)
  Estimation/4(descending) -> DtcDesc/1, term_desc/1

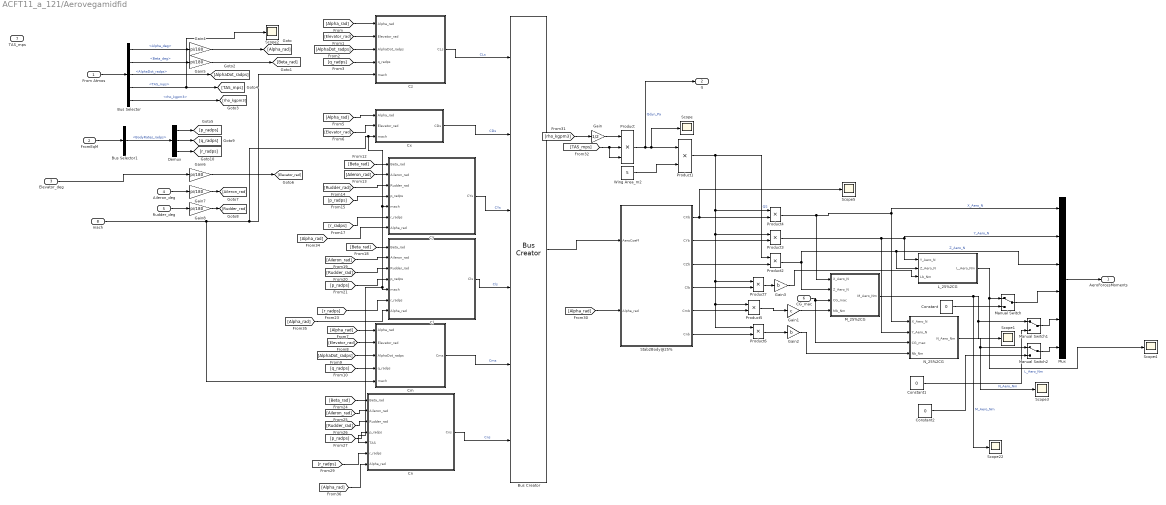
== system ACFT11_a_121/Aerovegamidfid ==
  From Atmos : Inport
  FromEqM : Inport  Port=2
  Elevator_deg : Inport  Port=3
  Aileron_deg : Inport  Port=4
  Rudder_deg : Inport  Port=5
  CG_mac : Inport  Port=6
  TAS_mps : Inport  Port=7
  mach : Inport  Port=8
  Bus Creator : BusCreator  Inputs=6
  Bus Selector : BusSelector  OutputSignals=Alpha_deg,Beta_deg,AlphaDot_radps,TAS_mps,rho_kgpm3
  Bus Selector1 : BusSelector  OutputSignals=BodyRates_radps
  CY : Subsystem
  Cl : Subsystem
  Cm : Subsystem
  Cn : Subsystem
  Constant : Constant  Value=0
  Constant1 : Constant  Value=0
  Constant2 : Constant  Value=0
  Cx : Subsystem
  Cz : Subsystem
  Demux : Demux  Outputs=3
  Gain : Gain  Gain=1/2
  Gain1 : Gain  Gain=c
  Gain2 : Gain  Gain=b
  Gain3 : Gain  Gain=b
  Gain{4..8} (5 alike) : Gain  Gain=pi/180
  L_25%2CG : Subsystem
  M_25%2CG : Subsystem
  Manual Switch : ManualSwitch
  Manual Switch1 : ManualSwitch
  Manual Switch2 : ManualSwitch
  Mux : Mux  Inputs=6
  N_25%2CG : Subsystem
  Product : Product  Inputs=3
  Product{1..7} (7 alike) : Product
  Scope{,1..5,22} (7 alike) : Scope
      Scope settings: ActiveDisplayYMinimum=-313.97579982351613  ActiveDisplayYMaximum=3159.0604943354219  DataLoggingVariableName=ScopeData10
      Scope1 settings: ActiveDisplayYMinimum=-297553.13250914251  ActiveDisplayYMaximum=806663.200823682  DataLoggingVariableName=ScopeData9
      Scope2 settings: ActiveDisplayYMinimum=167.07719132122796  ActiveDisplayYMaximum=315.34671758546926  DataLoggingVariableName=ScopeData19
      Scope22 settings: ActiveDisplayYMinimum=-6843.6751587663894  ActiveDisplayYMaximum=-269.53976890177387  DataLoggingVariableName=ScopeData45
      Scope3 settings: ActiveDisplayYMinimum=-929.591568641683  ActiveDisplayYMaximum=550.10636704149624  DataLoggingVariableName=ScopeData49
      Scope4 settings: DataLoggingVariableName=ScopeData50
      Scope5 settings: ActiveDisplayYMinimum=-0.0066232149368832746  ActiveDisplayYMaximum=-0.0066210769958273356  DataLoggingVariableName=ScopeData57
  Stab2Body@25% : Subsystem
  Wing Area_m2 : Constant  Value=S
  AeroForcesMoments : Outport
  q : Outport  Port=2
  wires:
  [Alpha_rad] -> Cn/7(Alpha_rad)
  [Alpha_rad] -> Cl/7(Alpha_rad)
  [Alpha_rad] -> CY/7(Alpha_rad)
  Bus Selector/5 -> [rho_kgpm3]  "<rho_kgpm3>"
  Bus Selector/4 -> Scope2/1, [TAS_mps]  "<TAS_mps>"
  N_25%2CG/1(N_Aero_Nm) -> Manual Switch2/1, Scope3/1  "N_Aero_Nm"
  Product/1 -> q/1, Scope/1, Product1/1  "Qdyn_Pa"
  [Aileron_rad] -> Cn/2(Aileron_rad)
  [p_radps] -> Cn/4(p_radps)
  Product5/1 -> Gain1/1
  [q_radps] -> Cm/4(q_radps)
  [AlphaDot_radps] -> Cm/3(AlphaDot_radps)
  CG_mac/1 -> M_25%2CG/3(CG_mac), N_25%2CG/3(CG_mac)
  Product4/1 -> M_25%2CG/1(X_Aero_N), N_25%2CG/1(X_Aero_N), Mux/1  "X_Aero_N"
  [Alpha_rad] -> Stab2Body@25%/2(Alpha_rad)
  Cn/1(Cns) -> Bus Creator/6  "Cns"
  Cz/1(CLs) -> Bus Creator/1  "CLs"
  L_25%2CG/1(L_Aero_Nm) -> Manual Switch/1, Scope4/1  "L_Aero_Nm"
  [Aileron_rad] -> CY/2(Aileron_rad)
  Cm/1(Cms) -> Bus Creator/5  "Cms"
  Gain3/1 -> L_25%2CG/3(Lb_Nm)
  Product6/1 -> Gain2/1
  M_25%2CG/1(M_Aero_Nm) -> Scope22/1, Scope1/1, Manual Switch1/1  "M_Aero_Nm"
  CY/1(CYs) -> Bus Creator/3  "CYs"
  [Rudder_rad] -> Cl/3(Rudder_rad)
  [r_radps] -> Cl/6(r_radps)
  Stab2Body@25%/5(Cmb) -> Product5/2
  Gain/1 -> Product/1
  Stab2Body@25%/3(CZb) -> Product2/2
  [TAS_mps] -> Product/2, Product/3
  Product3/1 -> N_25%2CG/2(Y_Aero_N), L_25%2CG/1(Y_Aero_N), Mux/2  "Y_Aero_N"
  [Aileron_rad] -> Cl/2(Aileron_rad)
  [rho_kgpm3] -> Gain/1
  Product7/1 -> Gain3/1
  Stab2Body@25%/4(Clb) -> Product7/2
  [Rudder_rad] -> Cn/3(Rudder_rad)
  Bus Creator/1 -> Stab2Body@25%/1(AeroCoeff)
  [r_radps] -> Cn/6(r_radps)
  Product2/1 -> M_25%2CG/2(Z_Aero_N), L_25%2CG/2(Z_Aero_N), Mux/3  "Z_Aero_N"
  Cx/1(CDs) -> Bus Creator/2  "CDs"
  Stab2Body@25%/6(Cnb) -> Product6/2
  Product1/1 -> Product4/1, Product5/1, Product6/1, Product7/1, Product3/1, Product2/1  "QS"
  Gain2/1 -> N_25%2CG/4(Nb_Nm)
  Stab2Body@25%/1(CXb) -> Scope5/1, Product4/2
  Cl/1(Cls) -> Bus Creator/4  "Cls"
  Wing Area_m2/1 -> Product1/2
  [r_radps] -> CY/6(r_radps)
  [Beta_rad] -> CY/1(Beta_rad)
  [Rudder_rad] -> CY/3(Rudder_rad)
  [Beta_rad] -> Cn/1(Beta_rad)
  [Beta_rad] -> Cl/1(Beta_rad)
  Gain1/1 -> M_25%2CG/4(Mb_Nm)
  [p_radps] -> Cl/4(p_radps)
  Stab2Body@25%/2(CYb) -> Product3/2
  [p_radps] -> CY/4(p_radps)
  Mux/1 -> AeroForcesMoments/1
  Gain5/1 -> [Beta_rad]
  Gain4/1 -> [Alpha_rad]
  Rudder_deg/1 -> Gain8/1
  Bus Selector/3 -> [AlphaDot_radps]  "<AlphaDot_radps>"
  [Elevator_rad] -> Cm/2(Elevator_rad)
  [Alpha_rad] -> Cm/1(Alpha_rad)
  [Elevator_rad] -> Cz/2(Elevator_rad)
  Elevator_deg/1 -> Gain6/1
  [Alpha_rad] -> Cz/1(Alpha_rad)
  [Elevator_rad] -> Cx/2(Elevator_rad)
  Gain8/1 -> [Rudder_rad]
  [Alpha_rad] -> Cx/1(Alpha_rad)
  [q_radps] -> Cz/4(q_radps)
  Bus Selector/2 -> Gain5/1  "<Beta_deg>"
  Gain7/1 -> [Aileron_rad]
  Aileron_deg/1 -> Gain7/1
  Demux/2 -> [q_radps]
  Demux/1 -> [p_radps]
  Gain6/1 -> [Elevator_rad]
  Demux/3 -> [r_radps]
  [AlphaDot_radps] -> Cz/3(AlphaDot_radps)
  From Atmos/1 -> Bus Selector/1
  Bus Selector/1 -> Gain4/1  "<Alpha_deg>"
  FromEqM/1 -> Bus Selector1/1
  Bus Selector1/1 -> Demux/1  "<BodyRates_radps>"
  Manual Switch/1 -> Mux/4
  Constant/1 -> Manual Switch/2
  Constant1/1 -> Manual Switch1/2
  Constant2/1 -> Manual Switch2/2
  Manual Switch1/1 -> Mux/5
  Manual Switch2/1 -> Mux/6
  mach/1 -> Cm/5(mach), Cz/5(mach), Cl/5(mach), Cn/5(TAS), CY/5(mach), Cx/3(mach)

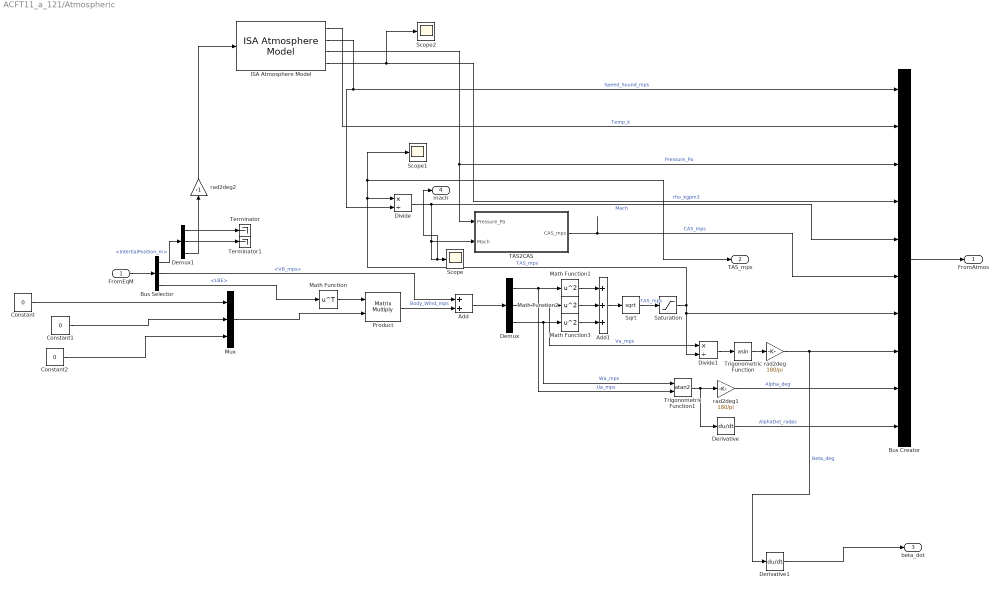
== system ACFT11_a_121/Atmospheric ==
  FromEqM : Inport
  Add : Sum
  Add1 : Sum  Inputs=+++
  Bus Creator : BusCreator  Inputs=10
  Bus Selector : BusSelector  OutputSignals=IntertialPosition_m,VB_mps,LBE
  Constant : Constant  Value=0
  Constant1 : Constant  Value=0
  Constant2 : Constant  Value=0
  Demux : Demux  Outputs=3
  Demux1 : Demux  Outputs=3
  Derivative : Derivative
  Derivative1 : Derivative
  Divide : Product  Inputs=*/
  Divide1 : Product  Inputs=*/
  ISA Atmosphere Model : aerolibatmos2/ISA Atmosphere Model  useExtended=on  action=None  custom=off  viscosityOut=off  g=9.80665  gamma=1.4  R=287.0531  L=0.0065  h_trop=11000  h_strat=20000  rho0=1.225  P0=101325  T0=288.15  h0=0  S=110.4  Tref=273.15  muref=1.716e-5
  Math Function : Math  Operator=transpose  SignedPower=on
  Math Function1 : Math  Operator=square  SignedPower=on
  Math Function2 : Math  Operator=square  SignedPower=on
  Math Function3 : Math  Operator=square  SignedPower=on
  Mux : Mux  Inputs=3
  Product : Product  Multiplication=Matrix(*)
  Saturation : Saturate  UpperLimit=inf  LowerLimit=1
  Scope : Scope
      settings: ActiveDisplayYMinimum=0.013245678240824399  ActiveDisplayYMaximum=3.7817118557135587  DataLoggingVariableName=ScopeData3
  Scope1 : Scope
      settings: ActiveDisplayYMinimum=90.384414191314278  ActiveDisplayYMaximum=989.75569914751316  YLabel=TAS(m/sec)
  Scope2 : Scope
      settings: ActiveDisplayYMinimum=0.38416  ActiveDisplayYMaximum=0.48694  DataLoggingVariableName=ScopeData10
  Sqrt : Sqrt
  TAS2CAS : Subsystem
  Terminator : Terminator
  Terminator1 : Terminator
  Trigonometric Function : Trigonometry  Operator=asin
  Trigonometric Function1 : Trigonometry  Operator=atan2
  rad2deg : Gain  Gain=180/pi
  rad2deg1 : Gain  Gain=180/pi
  rad2deg2 : Gain  Gain=-1
  FromAtmos : Outport
  TAS_mps : Outport  Port=2
  beta_dot : Outport  Port=3
  mach : Outport  Port=4
  wires:
  rad2deg/1 -> Derivative1/1, Bus Creator/8  "Beta_deg"
  Math Function3/1 -> Add1/3
  Add1/1 -> Sqrt/1
  Math Function1/1 -> Add1/1
  Demux/2 -> Math Function2/1, Divide1/1  "Va_mps"
  Demux/3 -> Math Function3/1, Trigonometric Function1/1  "Wa_mps"
  Divide1/1 -> Trigonometric Function/1
  Trigonometric Function/1 -> rad2deg/1
  Math Function2/1 -> Add1/2
  Demux/1 -> Math Function1/1, Trigonometric Function1/2  "Ua_mps"
  Add/1 -> Demux/1
  Demux1/3 -> rad2deg2/1
  TAS2CAS/1(CAS_mps) -> Bus Creator/6  "CAS_mps"
  Product/1 -> Add/2  "Body_Wind_mps"
  Mux/1 -> Product/2
  Math Function/1 -> Product/1
  Sqrt/1 -> Saturation/1  "TAS_mps"
  FromEqM/1 -> Bus Selector/1
  Divide/1 -> Bus Creator/5, mach/1, Scope/1, TAS2CAS/2(Mach)  "Mach"
  ISA Atmosphere Model/3 -> Bus Creator/3, TAS2CAS/1(Pressure_Pa)  "Pressure_Pa"
  ISA Atmosphere Model/1 -> Bus Creator/2  "Temp_k"
  ISA Atmosphere Model/2 -> Bus Creator/1, Divide/2  "Speed_Sound_mps"
  ISA Atmosphere Model/4 -> Scope2/1, Bus Creator/4  "rho_kgpm3"
  rad2deg1/1 -> Bus Creator/9  "Alpha_deg"
  Bus Creator/1 -> FromAtmos/1
  Trigonometric Function1/1 -> rad2deg1/1, Derivative/1
  Derivative/1 -> Bus Creator/10  "AlphaDot_radps"
  Bus Selector/3 -> Math Function/1  "<LBE>"
  Bus Selector/2 -> Add/1  "<VB_mps>"
  Bus Selector/1 -> Demux1/1  "<IntertialPosition_m>"
  Demux1/1 -> Terminator/1
  Demux1/2 -> Terminator1/1
  rad2deg2/1 -> ISA Atmosphere Model/1
  Saturation/1 -> TAS_mps/1, Scope1/1, Divide/1, Bus Creator/7, Divide1/2  "TAS_mps"
  Derivative1/1 -> beta_dot/1
  Constant/1 -> Mux/1
  Constant1/1 -> Mux/2
  Constant2/1 -> Mux/3

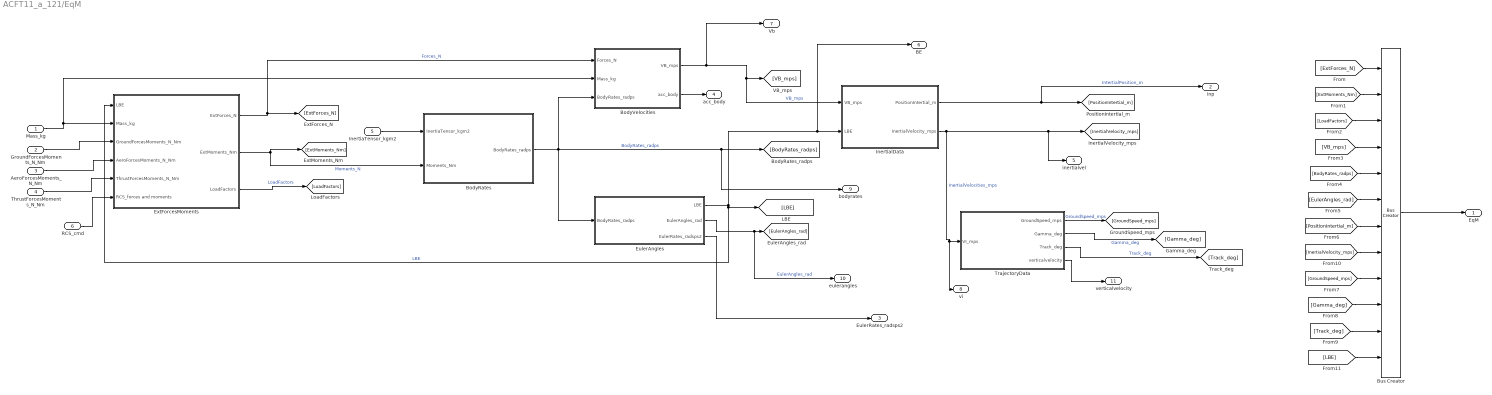
== system ACFT11_a_121/EqM ==
  Mass_kg : Inport
  GroundForcesMoments_N_Nm : Inport  Port=2
  AeroForcesMoments_N_Nm : Inport  Port=3
  ThrustForcesMoments_N_Nm : Inport  Port=4
  InertiaTensor_kgm2 : Inport  Port=5
  RCS_cmd : Inport  Port=6
  BodyRates : Subsystem
  BodyVelocities : Subsystem
  Bus Creator : BusCreator  Inputs=12
  EulerAngles : Subsystem
  ExtForcesMoments : Subsystem
  InertialData : Subsystem
  TrajectoryData : Subsystem
  EqM : Outport
  inp : Outport  Port=2
  EulerRates_radsps2 : Outport  Port=3
  acc_body : Outport  Port=4
  inertialvel : Outport  Port=5
  BE : Outport  Port=6
  Vb : Outport  Port=7
  vi : Outport  Port=8
  bodyrates : Outport  Port=9
  eulerangles : Outport  Port=10
  verticalvelocity : Outport  Port=11
  wires:
  [PositionIntertial_m] -> Bus Creator/7
  [EulerAngles_rad] -> Bus Creator/6
  [BodyRates_radps] -> Bus Creator/5
  [VB_mps] -> Bus Creator/4
  [ExtForces_N] -> Bus Creator/1
  Bus Creator/1 -> EqM/1
  [Track_deg] -> Bus Creator/11
  [ExtMoments_Nm] -> Bus Creator/2
  [Gamma_deg] -> Bus Creator/10
  [GroundSpeed_mps] -> Bus Creator/9
  TrajectoryData/1(GroundSpeed_mps) -> [GroundSpeed_mps]  "GroundSpeed_mps"
  EulerAngles/2(EulerAngles_rad) -> eulerangles/1, [EulerAngles_rad]  "EulerAngles_rad"
  TrajectoryData/3(Track_deg) -> [Track_deg]  "Track_deg"
  TrajectoryData/2(Gamma_deg) -> [Gamma_deg]  "Gamma_deg"
  AeroForcesMoments_N_Nm/1 -> ExtForcesMoments/4(AeroForcesMoments_N_Nm)
  ExtForcesMoments/3(LoadFactors) -> [LoadFactors]  "LoadFactors"
  Mass_kg/1 -> ExtForcesMoments/2(Mass_kg), BodyVelocities/2(Mass_kg)
  ExtForcesMoments/1(ExtForces_N) -> BodyVelocities/1(Forces_N), [ExtForces_N]  "Forces_N"
  BodyVelocities/1(VB_mps) -> Vb/1, InertialData/1(VB_mps), [VB_mps]  "VB_mps"
  EulerAngles/1(LBE) -> [LBE], ExtForcesMoments/1(LBE), BE/1, InertialData/2(LBE)  "LBE"
  GroundForcesMoments_N_Nm/1 -> ExtForcesMoments/3(GroundForcesMoments_N_Nm)
  ThrustForcesMoments_N_Nm/1 -> ExtForcesMoments/5(ThrustForcesMoments_N_Nm)
  BodyRates/1(BodyRates_radps) -> BodyVelocities/3(BodyRates_radps), EulerAngles/1(BodyRates_radps), bodyrates/1, [BodyRates_radps]  "BodyRates_radps"
  InertiaTensor_kgm2/1 -> BodyRates/1(InertiaTensor_kgm2)
  ExtForcesMoments/2(ExtMoments_Nm) -> [ExtMoments_Nm], BodyRates/2(Moments_Nm)  "Moments_N"
  [InertialVelocity_mps] -> Bus Creator/8
  [LoadFactors] -> Bus Creator/3
  InertialData/2(InertialVelocity_mps) -> vi/1, TrajectoryData/1(VI_mps), inertialvel/1, [InertialVelocity_mps]  "InertialVelocities_mps"
  InertialData/1(PositionIntertial_m) -> inp/1, [PositionIntertial_m]  "IntertialPosition_m"
  [LBE] -> Bus Creator/12
  EulerAngles/3(EulerRates_radsps2) -> EulerRates_radsps2/1
  BodyVelocities/2(acc_body) -> acc_body/1
  TrajectoryData/4(verticalvelocity) -> verticalvelocity/1
  RCS_cmd/1 -> ExtForcesMoments/6(RCS_forces and moments)

== system ACFT11_a_121/Estimation ==
  V : Inport
  rho : Inport  Port=2
  alt : Inport  Port=3
  gamma_deg : Inport  Port=4
  mach : Inport  Port=5
  E_sum : Sum
  Vsq : Product  Inputs=**
  Vz_calc : Product  Inputs=**
  desc_cmp : simulink/Logic and Bit Operations/Compare To Constant  relop=<  const=0  OutDataTypeStr=boolean
  gam_d2r : Gain  Gain=pi/180
  half : Gain  Gain=0.5
  ke_gain : Gain  Gain=1/(2*FCS_g)
  m_hi : simulink/Logic and Bit Operations/Compare To Constant  relop=<=  const=FCS_relight_M_hi  OutDataTypeStr=boolean
  m_lo : simulink/Logic and Bit Operations/Compare To Constant  relop=>=  const=FCS_relight_M_lo  OutDataTypeStr=boolean
  q_ok : simulink/Logic and Bit Operations/Compare To Constant  relop=>=  const=FCS_relight_qbar  OutDataTypeStr=boolean
  relight_and : Logic  Inputs=3  IconShape=distinctive  AllPortsSameDT=off  OutDataTypeStr=boolean
  rhoV2 : Product  Inputs=**
  sin_gam : Trigonometry
  E_spec : Outport
  qbar : Outport  Port=2
  Vz : Outport  Port=3
  descending : Outport  Port=4
  relight_ok : Outport  Port=5
  wires:
  relight_and/1 -> relight_ok/1
  q_ok/1 -> relight_and/3
  m_hi/1 -> relight_and/2
  m_lo/1 -> relight_and/1
  mach/1 -> m_lo/1, m_hi/1
  desc_cmp/1 -> descending/1
  Vz_calc/1 -> desc_cmp/1, Vz/1
  sin_gam/1 -> Vz_calc/2
  gam_d2r/1 -> sin_gam/1
  gamma_deg/1 -> gam_d2r/1
  E_sum/1 -> E_spec/1
  alt/1 -> E_sum/1
  ke_gain/1 -> E_sum/2
  half/1 -> qbar/1, q_ok/1
  rhoV2/1 -> half/1
  rho/1 -> rhoV2/2
  Vsq/1 -> rhoV2/1, ke_gain/1
  V/1 -> Vsq/2, Vsq/1, Vz_calc/1

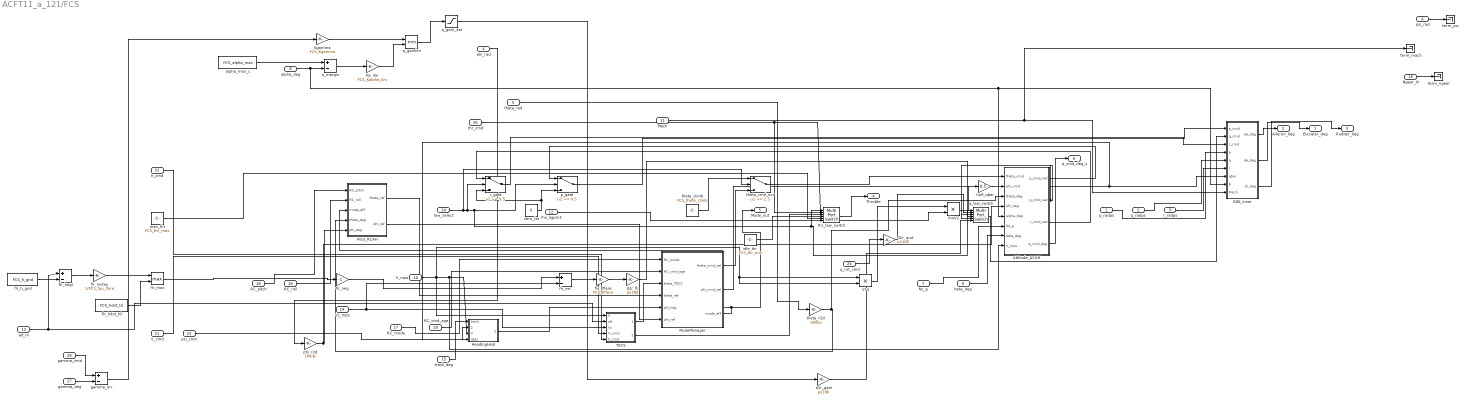
== system ACFT11_a_121/FCS ==
  p_radps : Inport
  q_radps : Inport  Port=2
  r_radps : Inport  Port=3
  phi_rad : Inport  Port=4
  theta_rad : Inport  Port=5
  psi_rad : Inport  Port=6
  Nz_g : Inport  Port=7
  alpha_deg : Inport  Port=8
  beta_deg : Inport  Port=9
  V_mps : Inport  Port=10
  Mach : Inport  Port=11
  rho_kgpm3 : Inport  Port=12
  alt_m : Inport  Port=13
  Vz_mps : Inport  Port=14
  track_deg : Inport  Port=15
  Ngear_N : Inport  Port=16
  RC_mode : Inport  Port=17
  RC_pitch : Inport  Port=18
  RC_roll : Inport  Port=19
  RC_cmd_age : Inport  Port=20
  V_cmd : Inport  Port=21
  h_cmd : Inport  Port=22
  psi_cmd : Inport  Port=23
  law_select : Inport  Port=24
  q_rot_cmd : Inport  Port=25
  thr_cmd : Inport  Port=26
  gamma_deg : Inport  Port=27
  gamma_cmd : Inport  Port=28
  Attitude_ACAH : Subsystem
  HeadingHold : Subsystem
  INDI_Inner : Subsystem
  Ka_lim : Gain  Gain=FCS_Kalpha_lim
  Kgamma : Gain  Gain=FCS_Kgamma
  ModeManager : Subsystem
  Pilot_RCAH : Subsystem
  TECS : Subsystem
  Vsq : Product  Inputs=**
  a_margin : Sum  Inputs=+-
  alpha_max_c : Constant  Value=FCS_alpha_max
  d2r_flr : Gain  Gain=pi/180
  d2r_gam : Gain  Gain=pi/180
  d2r_qrot : Gain  Gain=pi/180
  flr_Kflare : Gain  Gain=FCS_Kflare
  flr_err : Sum  Inputs=|+-
  flr_h_gnd : Constant  Value=FCS_h_gnd
  flr_hagl : Sum  Inputs=|+-
  flr_hdot_td : Constant  Value=FCS_hdot_td
  flr_invtau : Gain  Gain=1/FCS_tau_flare
  flr_max : MinMax  Function=max  Inputs=2
  flr_neg : Gain  Gain=-1
  gamma_err : Sum  Inputs=+-
  half_qbar : Gain  Gain=0.5
  idle_thr : Constant  Value=FCS_thr_min
  max_thr : Constant  Value=FCS_thr_max
  p_gate : Switch  Threshold=0.5  SaturateOnIntegerOverflow=off  InputSameDT=off
  phi_r2d : Gain  Gain=180/pi
  q_gam_sat : Saturate  UpperLimit=FCS_q_max  LowerLimit=-FCS_q_max
  q_gamlim : MinMax  Inputs=2
  q_law_switch : MultiPortSwitch  DataPortOrder=Zero-based contiguous  Inputs=5  zeroidx=on  SaturateOnIntegerOverflow=off  InputSameDT=off
  r_gate : Switch  Threshold=0.5  SaturateOnIntegerOverflow=off  InputSameDT=off
  rhoV2 : Product  Inputs=**
  term_mach : Terminator
  term_ngear : Terminator
  term_psi : Terminator
  theta_climb : Constant  Value=FCS_theta_climb
  theta_cmd_ovr : Switch  Threshold=2.5  SaturateOnIntegerOverflow=off  InputSameDT=off
  theta_r2d : Gain  Gain=180/pi
  thr_law_switch : MultiPortSwitch  DataPortOrder=Zero-based contiguous  Inputs=5  zeroidx=on  SaturateOnIntegerOverflow=off  InputSameDT=off
  zero_lat : Constant  Value=0
  Elevator_deg : Outport
  Aileron_deg : Outport  Port=2
  Rudder_deg : Outport  Port=3
  Throttle : Outport  Port=4
  Mode_out : Outport  Port=5
  q_cmd_deg_s : Outport  Port=6
  wires:
  INDI_Inner/3(dr_deg) -> Rudder_deg/1
  INDI_Inner/2(de_deg) -> Elevator_deg/1
  INDI_Inner/1(da_deg) -> Aileron_deg/1
  Attitude_ACAH/4(q_cmd_deg) -> q_cmd_deg_s/1
  beta_deg/1 -> Attitude_ACAH/7(beta_deg)
  Nz_g/1 -> Attitude_ACAH/6(Nz_g)
  ModeManager/2(phi_cmd_sel) -> Attitude_ACAH/2(phi_cmd)
  RC_cmd_age/1 -> ModeManager/2(RC_cmd_age)
  RC_mode/1 -> ModeManager/1(RC_mode)
  Pilot_RCAH/2(phi_ref) -> ModeManager/6(phi_ref)
  Pilot_RCAH/1(theta_ref) -> ModeManager/4(theta_ref)
  ModeManager/3(mode_eff) -> Pilot_RCAH/3(mode_eff), Mode_out/1
  RC_roll/1 -> Pilot_RCAH/2(RC_roll)
  RC_pitch/1 -> Pilot_RCAH/1(RC_pitch)
  HeadingHold/1(phi_cmd) -> ModeManager/5(phi_hdg)
  track_deg/1 -> HeadingHold/1(track)
  TECS/1(theta_cmd) -> ModeManager/3(theta_TECS)
  r_radps/1 -> INDI_Inner/6(r)
  q_radps/1 -> INDI_Inner/5(q)
  p_radps/1 -> INDI_Inner/4(p)
  phi_rad/1 -> phi_r2d/1
  rhoV2/1 -> half_qbar/1
  half_qbar/1 -> HeadingHold/4(qbar), INDI_Inner/7(qbar)
  phi_r2d/1 -> Pilot_RCAH/5(phi_deg), Attitude_ACAH/4(phi_deg)
  rho_kgpm3/1 -> rhoV2/2
  Ngear_N/1 -> term_ngear/1
  psi_rad/1 -> term_psi/1
  thr_law_switch/1 -> Throttle/1
  q_law_switch/1 -> INDI_Inner/2(q_cmd)
  TECS/2(Throttle) -> thr_law_switch/3
  Attitude_ACAH/2(q_cmd_rad) -> q_law_switch/5, q_law_switch/3
  idle_thr/1 -> thr_law_switch/4
  d2r_qrot/1 -> q_law_switch/2
  q_rot_cmd/1 -> d2r_qrot/1
  psi_cmd/1 -> HeadingHold/2(psi_cmd)
  h_cmd/1 -> TECS/5(h_cmd)
  V_cmd/1 -> TECS/4(V_cmd)
  theta_r2d/1 -> Attitude_ACAH/3(theta_deg), Pilot_RCAH/4(theta_deg)
  theta_rad/1 -> theta_r2d/1
  theta_cmd_ovr/1 -> Attitude_ACAH/1(theta_cmd)
  ModeManager/1(theta_cmd_sel) -> theta_cmd_ovr/3
  theta_climb/1 -> theta_cmd_ovr/1
  max_thr/1 -> thr_law_switch/5
  r_gate/1 -> INDI_Inner/3(r_cmd)
  Attitude_ACAH/3(r_cmd_rad) -> r_gate/1
  p_gate/1 -> INDI_Inner/1(p_cmd)
  zero_lat/1 -> r_gate/3, p_gate/3
  Attitude_ACAH/1(p_cmd_rad) -> p_gate/1
  law_select/1 -> thr_law_switch/1, q_law_switch/1, p_gate/2, r_gate/2, theta_cmd_ovr/2
  d2r_gam/1 -> q_law_switch/6
  gamma_deg/1 -> gamma_err/2
  gamma_cmd/1 -> gamma_err/1
  thr_cmd/1 -> thr_law_switch/6, thr_law_switch/2
  Mach/1 -> INDI_Inner/9(Mach), term_mach/1
  q_gamlim/1 -> q_gam_sat/1
  Ka_lim/1 -> q_gamlim/2
  Kgamma/1 -> q_gamlim/1
  a_margin/1 -> Ka_lim/1
  alpha_max_c/1 -> a_margin/1
  alpha_deg/1 -> Attitude_ACAH/5(alpha_deg), INDI_Inner/8(alpha_deg), a_margin/2
  gamma_err/1 -> Kgamma/1
  q_gam_sat/1 -> d2r_gam/1
  flr_Kflare/1 -> d2r_flr/1
  flr_err/1 -> flr_Kflare/1
  flr_neg/1 -> flr_err/1
  flr_max/1 -> flr_neg/1
  flr_hdot_td/1 -> flr_max/2
  flr_invtau/1 -> flr_max/1
  flr_hagl/1 -> flr_invtau/1
  flr_h_gnd/1 -> flr_hagl/2
  d2r_flr/1 -> q_law_switch/4
  alt_m/1 -> flr_hagl/1, TECS/2(alt)
  Vz_mps/1 -> flr_err/2, TECS/3(Vz)
  V_mps/1 -> HeadingHold/3(V), Attitude_ACAH/8(V_mps), Vsq/1, Vsq/2, TECS/1(V)
  Vsq/1 -> rhoV2/1

== system ACFT11_a_121/Landing Gear ==
  EulerAngles_rad : Inport
  VB_mps : Inport  Port=2
  BodyRates_radps : Inport  Port=3
  pos_NED_m : Inport  Port=4
  mass_kg : Inport  Port=5
  mu_cmd : Inport  Port=6
  LandingGear_FCN : MATLAB Function  TreatAsAtomicUnit=on
  GndForces_N_Nm : Outport
  N_total_N : Outport  Port=2
  N_gears_N : Outport  Port=3
  wires:
  ? -> ?
  EulerAngles_rad/1 -> LandingGear_FCN/1(EulerAngles_rad)
  VB_mps/1 -> LandingGear_FCN/2(VB_mps)
  BodyRates_radps/1 -> LandingGear_FCN/3(BodyRates_radps)
  pos_NED_m/1 -> LandingGear_FCN/4(pos_NED_m)
  mass_kg/1 -> LandingGear_FCN/5(mass_kg)
  LandingGear_FCN/1(GndForces) -> GndForces_N_Nm/1
  LandingGear_FCN/2(N_total) -> N_total_N/1
  LandingGear_FCN/3(N_gears) -> N_gears_N/1
  mu_cmd/1 -> LandingGear_FCN/6(mu_cmd)

== system ACFT11_a_121/Propulsion ==
  FromAtmos : Inport
  Throttle : Inport  Port=2
  Mach : Inport  Port=3
  Bus Selector : BusSelector  OutputSignals=rho_kgpm3
  PropulsionFCN : MATLAB Function  TreatAsAtomicUnit=on
  Sel_Forces : Selector  InputPortWidth=7  IndexOptions=Index vector (dialog)  Indices=[1 2 3 4 5 6]  OutputSizes=1
  Sel_Thrust : Selector  InputPortWidth=7  IndexOptions=Index vector (dialog)  Indices=[7]  OutputSizes=1
  Engine_Forces_and Moments : Outport
  Thrust_N : Outport  Port=2
  wires:
  FromAtmos/1 -> Bus Selector/1
  Mach/1 -> PropulsionFCN/1(Mach)
  Bus Selector/1 -> PropulsionFCN/2(rho_kgpm3)  "<rho_kgpm3>"
  Throttle/1 -> PropulsionFCN/3(Throttle)
  PropulsionFCN/1(y) -> Sel_Forces/1, Sel_Thrust/1
  Sel_Forces/1 -> Engine_Forces_and Moments/1
  Sel_Thrust/1 -> Thrust_N/1

== system ACFT11_a_121/aerospike ==
  Manual Switch1 : ManualSwitch
  Scope1 : Scope
      settings: ActiveDisplayYMinimum=711.4  ActiveDisplayYMaximum=2711.4  DataLoggingVariableName=ScopeData8
  TotalWeight full : Constant  Value=24000
  TotalWeightempty : Constant  Value=10800
  net mass : Outport
  wires:
  TotalWeight full/1 -> Manual Switch1/1
  Manual Switch1/1 -> net mass/1, Scope1/1
  TotalWeightempty/1 -> Manual Switch1/2
